simulink library "Brakes_Lib"  (R2025a)
settings: Solver=ode45  StartTime=0.0  StopTime=10.0  RelTol=1e-3  EnableMultiTasking=on
undefined symbols (not defined in the file): WT_Params
libraries: fl_lib x5, nesl_utility x2, sdl_lib x1
Description:
  | Copyright 2009-2025 The MathWorks, Inc. MathWorks, Inc.
settings Model: Creator=smiller  LastModifiedBy=smiller
settings SolverCC: AlgebraicLoopSolver=TrustRegion
settings DataIOCC: LimitDataPoints=on  SaveFormat=Array  SignalLoggingSaveFormat=ModelDataLogs  ReturnWorkspaceOutputs=off
settings OptimizationCC: ReuseModelBlockBuffer=off  ExpressionDepthLimit=2147483647.0  LifeSpan=inf
settings DebuggingCC: UnderspecifiedInitializationDetection=Classic  MergeDetectMultiDrivingBlocksExec=none  SolverPrmCheckMsg=warning  FcnCallInpInsideContextMsg=warning  UnconnectedInputMsg=warning  UnconnectedOutputMsg=warning  UnconnectedLineMsg=warning  AllowSymbolicDim=off  StateNameClashWarn=warning  PregeneratedLibrarySubsystemCodeDiagnostic=none  SFUnexpectedBacktrackingDiag=warning  SFNoUnconditionalDefaultTransitionDiag=warning  SFExecutionAtInitializationDiag=none  ArithmeticOperatorsInVariantConditions=warning
settings HardwareCC: ProdBitPerPointer=32.0  ProdBitPerSizeT=32.0  ProdBitPerPtrDiffT=32.0  ProdLargestAtomicFloat=None  ProdIntDivRoundTo=Undefined  ProdEndianess=Unspecified  ProdWordSize=32.0  ProdHWDeviceType=32-bit Generic
settings ModelReferenceCC: EnableRefExpFcnMdlSchedulingChecks=on  PropagateSignalLabelsOutOfModel=off
settings SFSimCC: SimUseLocalCustomCode=off  CustomCodeUndefinedFunction=UseInterfaceOnly
settings RTWCC: RTWUseLocalCustomCode=off  GPUComputeCapability=3.5  DLArmComputeVersion=19.05
settings CodeAppCC: StateflowObjectComments=on
settings GRTTargetCC: TargetLangStandard=C89/C90 (ANSI)  CombineOutputUpdateFcns=off  GRTInterface=on
settings ConfigComp: CovMetricSettings=dw  CovSaveCumulativeToWorkspaceVar=on  CovSaveSingleToWorkspaceVar=on  CovExternalEMLEnable=off  CovSFcnEnable=off

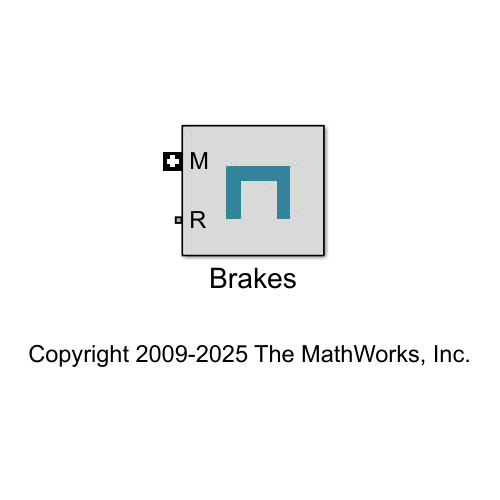
[thumbnail: Simulink's stored preview of the top-level diagram]
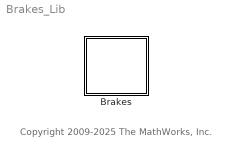
== system Brakes_Lib ==
  note: Copyright 2009-2025 The MathWorks, Inc.
  Brakes : Subsystem
      mask Display: image('Brakes_IMAGE.jpg');

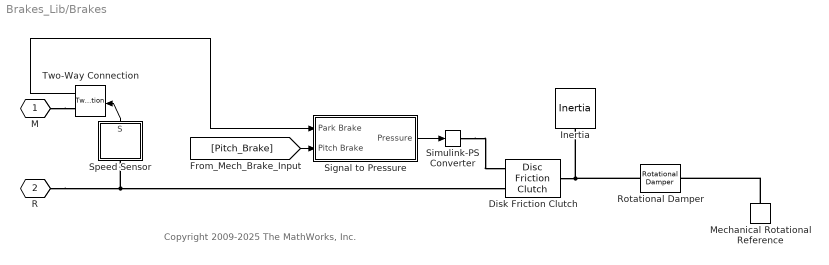
== system Brakes_Lib/Brakes ==
  note: Copyright 2009-2025 The MathWorks, Inc.
  Disk Friction Clutch : sdl_lib/Clutches/Disc Friction Clutch  geometry_model=1  r_eff=WT_Params.Brakes.torque_radius m  d_o=150 mm  d_i=100 mm  nS=WT_Params.Brakes.num_friction_surfaces  piston_area=WT_Params.Brakes.piston_area m^2  unidirectional=0  friction_model=1  mu_w_vector=[1 1e8] rad/s  temperature_TLU=[280.0, 300.0, 320.0] K  mu_static=WT_Params.Brakes.static_friction_coeff  mu_static_vector=[0.4, 0.38, 0.36]  mu_coulomb=WT_Params.Brakes.kinetic_friction_coeff  mu_coulomb_vector=[0.3 0.001]  mu_coulomb_temp_vector=[0.3, 0.28, 0.25]  mu_coulomb_matrix=[0.34, 0.32, 0.3; 0.3, 0.28, 0.25; 0.25, 0.2, 0.15]  mu_interp_method=1  mu_extrap_method=1  d_f=1  w_tol=WT_Params.Brakes.clutch_vel_tol rad/s  pressure_min=WT_Params.Brakes.threshold_pressure Pa  mu_visc=0 N*m/(rad/s)  initial_state_locked=1  thermal_mass=25 kJ/K  T_init=300 K
      settings: InternalSimscapePortConfiguration="{\"Bottom\":[],\"Left\":[{\"id\":\"P\",\"label\":\"P\",\"type\":\"input\"},{\"id\":\"B\",\"label\":\"B\",\"type\":\"foundation.mechanical.rotational.rotational\"}],\"Right\":[{\"id\":\"F\",\"label\":\"F\",\"type\":\"foundation.mechanical.rotational.rotational\"}],\"Top\":[]}"
  Inertia : fl_lib/Mechanical/Rotational Elements/Inertia  inertia=WT_Params.Brakes.inertia_housing kg*m^2  num_ports=foundation.enum.numPorts2.one  w_specify=on  w_priority=High  w=0 rad/s  w_nominal_specify=off  w_nominal_value=1  w_nominal_unit=rad/s  t_specify=off  t_priority=High  t=0 N*m  t_nominal_specify=off  t_nominal_value=1  t_nominal_unit=N*m
  Mechanical Rotational Reference : fl_lib/Mechanical/Rotational Elements/Mechanical Rotational Reference
  Rotational Damper : fl_lib/Mechanical/Rotational Elements/Rotational Damper  D=WT_Params.Brakes.damping N*m/(rad/s)  w_specify=off  w_priority=High  w=0 rad/s  w_nominal_specify=off  w_nominal_value=1  w_nominal_unit=rad/s  t_specify=off  t_priority=High  t=0 N*m  t_nominal_specify=off  t_nominal_value=1  t_nominal_unit=N*m
  Signal to Pressure : Subsystem
  Simulink-PS Converter : nesl_utility/Simulink-PS Converter  PhysicalDomain=network_engine_domain  SubClassName=ps_input  LeftPortType=input  RightPortType=output  PseudoPeriodic=off  Frequencies=[]  NoiseDistribution=none  NoiseParameters=[]  Unit=1  AffineConversion=off  FilteringAndDerivatives=zero  SimscapeFilterOrder=1  InputFilterTimeConstant=0.005  UdotUserProvided=0
  Speed Sensor : Subsystem
      mask Display:
      | plot([149.600878633536;150.016472378793;150.47508104106;150.972287968219;151.50330478576;152.063017511447;152.646035805762;153.246744883819;153.859359588817;154.477980106257;155.096648782383;155.709407499646;156.310355056631;156.893703999851;157.453836360095;157.985357756531;158.483149347555;158.942417128023;159.358738098149;159.728102859405;160.046954227227;160.312221488639;160.521349974904;160.672325664379;160.763694578642;160.794576785101;160.764674871227;160.674276808796;160.524253180566;160.316048796087;160.051668777399;159.733659248606;159.365082815313;158.949489070056;158.490880407788;157.993673480629;157.462656663088;156.908284800231], [156.971389291536;157.430657072004;157.84697804213;158.216342803387;158.535194171208;158.80046143262;159.009589918885;159.16056560836;159.251934522623;159.282816729083;159.252914815208;159.162516752777;159.012493124547;158.804288740068;158.53990872138;158.221899192587;157.853322759294;157.437729014037;156.979120351769;156.48191342461;155.950896607069;155.391183881382;154.808165587067;154.20745650901;153.594841804012;152.976221286573;152.357552610446;151.744793893183;151.143846336199;150.560497392978;150.000365032735;149.468843636298;148.971052045274;148.511784264806;148.095463294681;147.726098533424;147.407247165603;147.144199990631])
      | plot([152.057635404444;152.93604260309;153.834625296826;154.744729643097;155.657590839533;156.564417533794;157.45647648909;158.325176690034;159.162152078811;159.959342124889;160.709069452336;161.404113777147;162.037781442523;162.603969882449;163.097226392739;163.512800643557;163.846690427691;164.095680203997;164.257372064819;164.330208829146;164.313489039122;164.27939575172], [142.228020686971;141.979030910664;141.817339049842;141.744502285515;141.761222075539;141.867337399197;142.061826307913;142.342815767178;142.707599694895;143.152665022428;143.673725527376;144.265763112236;144.923076131425;145.639334301243;146.40763966397;147.220593018964;148.070365181011;148.948772379657;149.847355073393;150.757459419663;151.6703206161;152.055850472277])
      | plot([116.468514315784;116.438789536125;116.349901463023;116.202706137216;115.998621130155;115.739611892022;115.42817282337;115.067303252679;114.660478551187;114.211616663162;113.725040373958;113.205435679231;112.657806656235;112.087427271827;111.499790591278;110.900555877058;110.29549408704;109.690432297022;109.091197582803;108.503560902254;107.933181517846;107.38555249485;106.865947800123;106.379371510919;105.930509622894;105.523684921402;105.162815350711;104.851376282059;104.592367043926;104.388282036865;104.241086711057;104.152198637956;104.122473858297;104.152198637956;104.241086711057;104.388282036865;104.592367043926;104.851376282059;105.162815350711;105.523684921402;105.930509622894;106.379371510919;106.865947800123;107.38555249485;107.933181517846;108.503560902254;109.091197582803;109.690432297022;110.29549408704;110.900555877058;111.499790591278;112.087427271827;112.657806656235;113.205435679231;113.725040373958;114.211616663162;114.660478551187;115.067303252679;115.42817282337;115.739611892022;115.998621130155;116.202706137216;116.349901463023;116.438789536125;116.468514315784;116.468514315784], [111.618284136057;111.013222346039;110.413987631819;109.826350951271;109.255971566862;108.708342543866;108.188737849139;107.702161559936;107.253299671911;106.846474970419;106.485605399728;106.174166331075;105.915157092943;105.711072085881;105.563876760074;105.474988686973;105.445263907313;105.474988686973;105.563876760074;105.711072085881;105.915157092943;106.174166331075;106.485605399728;106.846474970419;107.253299671911;107.702161559936;108.188737849139;108.708342543866;109.255971566862;109.826350951271;110.413987631819;111.013222346039;111.618284136057;112.223345926075;112.822580640295;113.410217320843;113.980596705252;114.528225728247;115.047830422975;115.534406712178;115.983268600203;116.390093301695;116.750962872386;117.062401941038;117.321411179171;117.525496186232;117.67269151204;117.761579585141;117.7913043648;117.761579585141;117.67269151204;117.525496186232;117.321411179171;117.062401941038;116.750962872386;116.390093301695;115.983268600203;115.534406712178;115.047830422975;114.528225728247;113.980596705252;113.410217320843;112.822580640295;112.223345926075;111.618284136057;111.618284136057])
      | plot([239.23602886498;238.828071429858;237.608127977604;235.587947230552;232.78698463364;229.232214987837;224.957872668068;220.005121927465;214.421660463109;208.261260061133;201.583248745024;194.451939414329;186.936010476274;179.107844435155;171.042830809261;162.818640088593;154.514475725591;146.210311362589;137.986120641921;129.921107016027;122.092940974909;114.577012036853;107.445702706158;100.76769139005;94.607290988073;89.0238295237172;84.0710787831142;79.7967364633452;76.2419668175427;73.4410042206305;71.4208234735788;70.2008800213248;69.7929225862026;70.2008800213248;71.4208234735788;73.4410042206306;76.2419668175428;79.7967364633454;84.0710787831144;89.0238295237174;94.6072909880733;100.76769139005;107.445702706159;114.577012036853;122.092940974909;129.921107016027;137.986120641921;146.210311362589;154.514475725591;162.818640088593;171.042830809261;179.107844435155;186.936010476274;194.451939414329;201.583248745024;208.261260061133;214.421660463109;220.005121927465;224.957872668068;229.232214987837;232.78698463364;235.587947230552;237.608127977604;238.828071429858;239.23602886498;239.23602886498], [155.774275772274;147.47628550917;139.258209428443;131.199192095207;123.376846251889;115.866505365088;108.740498123116;102.067451871182;95.9116316925529;90.3323215006612;85.3832531026163;81.1120887325275;77.5599620381344;74.7610819412943;72.742403187363;71.5233667562631;71.1157126352191;71.5233667562631;72.742403187363;74.7610819412943;77.5599620381345;81.1120887325275;85.3832531026164;90.3323215006612;95.9116316925529;102.067451871182;108.740498123116;115.866505365089;123.376846251889;131.199192095207;139.258209428443;147.47628550917;155.774275772274;164.072266035377;172.290342116104;180.34935944934;188.171705292658;195.682046179459;202.808053421432;209.481099673365;215.636919851994;221.216230043886;226.165298441931;230.43646281202;233.988589506413;236.787469603253;238.806148357184;240.025184788284;240.432838909328;240.025184788284;238.806148357184;236.787469603253;233.988589506413;230.43646281202;226.165298441931;221.216230043886;215.636919851994;209.481099673365;202.808053421432;195.682046179459;188.171705292658;180.34935944934;172.290342116105;164.072266035378;155.774275772274;155.774275772274])
      | plot([252.715889364481;252.243022716633;250.828976737403;248.487369462568;245.240751850236;241.120390602797;236.165967051481;230.425195003451;223.953361231755;216.812793033479;209.072257983804;200.806301666664;192.094529760025;183.020841389688;173.672621134841;164.139897466795;154.514475725591;144.889053984387;135.356330316341;126.008110061494;116.934421691157;108.222649784518;99.9566934673787;92.2161584177032;85.075590219427;78.6037564477313;72.8629843997015;67.9085608483856;63.7881996009461;60.5415819886144;58.199974713779;56.7859287345493;56.3130620867014;56.7859287345493;58.1999747137791;60.5415819886146;63.7881996009463;67.9085608483858;72.8629843997018;78.6037564477315;85.0755902194273;92.2161584177035;99.9566934673791;108.222649784519;116.934421691157;126.008110061494;135.356330316341;144.889053984387;154.514475725591;164.139897466796;173.672621134841;183.020841389688;192.094529760025;200.806301666664;209.072257983803;216.812793033479;223.953361231755;230.425195003451;236.165967051481;241.120390602797;245.240751850236;248.487369462568;250.828976737403;252.243022716633;252.715889364481;252.715889364481], [154.514475725591;144.895228084285;135.36861905618;126.026395093992;116.958526921455;108.252343066071;99.9916888376535;92.2561188521535;85.1201308772245;78.6524483779929;72.9153586725213;67.9641130708855;63.8463947748555;60.6018596625959;58.2617543808809;56.8486154228053;56.3760520890355;56.8486154228053;58.2617543808809;60.6018596625959;63.8463947748555;67.9641130708856;72.9153586725213;78.652448377993;85.1201308772246;92.2561188521536;99.9916888376536;108.252343066072;116.958526921455;126.026395093992;135.36861905618;144.895228084285;154.514475725591;164.133723366898;173.660332395002;183.002556357191;192.070424529728;200.776608385111;209.037262613529;216.772832599029;223.908820573958;230.37650307319;236.113592778661;241.064838380297;245.182556676327;248.427091788587;250.767197070302;252.180336028377;252.652899362147;252.180336028377;250.767197070301;248.427091788587;245.182556676327;241.064838380297;236.113592778661;230.37650307319;223.908820573958;216.772832599029;209.037262613529;200.776608385111;192.070424529728;183.002556357191;173.660332395002;164.133723366898;154.514475725592;154.514475725591])
      | plot([154.514475725591;129.948374815285;179.017586633563;154.514475725591], [240.369848906994;203.583687543869;203.583687543869;240.369848906994])
      | plot([105.382273904979;149.60125554353], [115.271704271436;156.971085816622])
      | plot([144.688035361469;144.688035361469], [152.057865634561;203.583687543869])
      | plot([164.277926087379;164.277926087379], [152.057865634561;203.583687543869])
      | plot([159.112745895982;159.616665914655], [149.60125554353;149.60125554353])
      | plot([115.208714269102;159.364705905318], [107.901873998344;149.60125554353])
      | plot([0;311.800511553884;311.800511553884;0;0], [311.800511553884;311.800511553884;0;0;311.800511553884])
      | ;
      | color('red');
      | port_label('LConn', 1,'R')
      | port_label('output', 1,'W')
  Two-Way Connection : TwoWayConnection
  M : PMIOPort  Tag=PMCPort  Side=Left
  R : PMIOPort  Tag=PMCPort  Port=2  Side=Left
  wires:
  Signal to Pressure/1(Pressure) -> Simulink-PS Converter/1
  Two-Way Connection/1 -> Signal to Pressure/1(Park Brake)
  Speed Sensor/1(S) -> Two-Way Connection/1
  [Pitch_Brake] -> Signal to Pressure/2(Pitch Brake)
  connections:
  Simulink-PS Converter/RConn1 -- Disk Friction Clutch/LConn1
  R/RConn1 -- Disk Friction Clutch/LConn2 -- Speed Sensor/LConn1
  M/RConn1 -- Two-Way Connection/RConn1
  Mechanical Rotational Reference/LConn1 -- Rotational Damper/RConn1
  Disk Friction Clutch/RConn1 -- Inertia/LConn1 -- Rotational Damper/LConn1

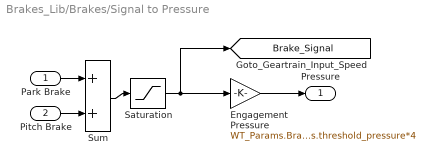
== system Brakes_Lib/Brakes/Signal to Pressure ==
  Park Brake : Inport
  Pitch Brake : Inport  Port=2
  Engagement Pressure : Gain  Gain=WT_Params.Brakes.threshold_pressure*4
  Saturation : Saturate  UpperLimit=1  LowerLimit=0  ZeroCross=off
  Sum : Sum
  Pressure : Outport  VectorParamsAs1DForOutWhenUnconnected=off
  tag scope: Brake_Signal=global
  wires:
  Sum/1 -> Saturation/1
  Saturation/1 -> Engagement Pressure/1, [Brake_Signal]
  Park Brake/1 -> Sum/1
  Engagement Pressure/1 -> Pressure/1
  Pitch Brake/1 -> Sum/2

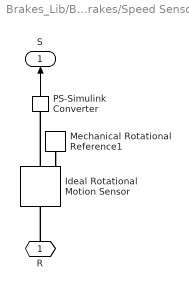
== system Brakes_Lib/Brakes/Speed Sensor ==
  Ideal Rotational Motion Sensor : fl_lib/Mechanical/Mechanical Sensors/Ideal Rotational Motion Sensor  reference=foundation.enum.MeasurementReference.difference  acceleration_port=false  velocity_port=true  position_port=true  wrap_angle=simscape.enum.onoff.off  offset=0 rad
  Mechanical Rotational Reference1 : fl_lib/Mechanical/Rotational Elements/Mechanical Rotational Reference
  PS-Simulink Converter : nesl_utility/PS-Simulink Converter  PhysicalDomain=network_engine_domain  SubClassName=ps_output  LeftPortType=input  RightPortType=output  PseudoPeriodic=off  Frequencies=[]  VectorFormat=1-D array  Unit=1  AffineConversion=off
  R : PMIOPort  Side=Left
  S : Outport  VectorParamsAs1DForOutWhenUnconnected=off
  wires:
  PS-Simulink Converter/1 -> S/1
  connections:
  Ideal Rotational Motion Sensor/RConn2 -- PS-Simulink Converter/LConn1
  R/RConn1 -- Ideal Rotational Motion Sensor/LConn1
  Mechanical Rotational Reference1/LConn1 -- Ideal Rotational Motion Sensor/RConn1
